simulink model "sc_1"  (R2024b)
settings: Solver=VariableStepAuto  StartTime=0.0  StopTime=10.0  RelTol=1e-3
settings Model: Creator=alex_  LastModifiedBy=alex_

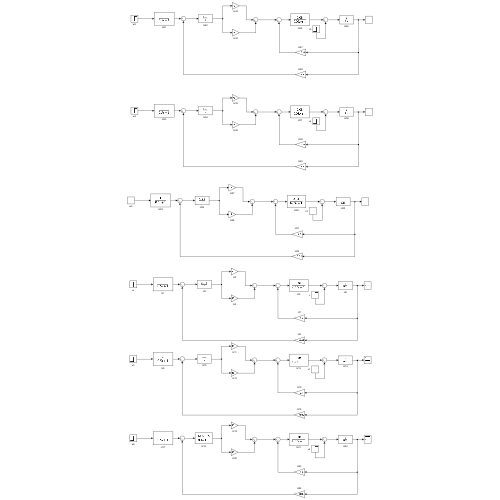
[thumbnail: Simulink's stored preview of the top-level diagram]
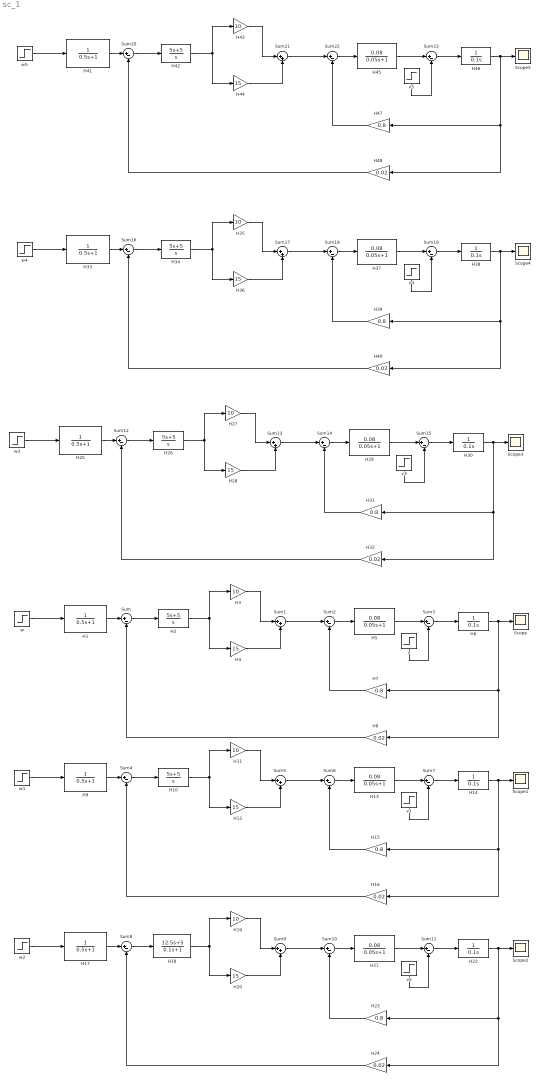
== system sc_1 ==
  H{1,9,17,25,33,41} (6 alike) : TransferFcn  Denominator=[0.5 1]
  H{2,10,26,34,42} (5 alike) : TransferFcn  Numerator=[5 5]  Denominator=[1 0]
  H{3,11,19,27,35,43} (6 alike) : Gain  Gain=10
  H{4,12,20,28,36,44} (6 alike) : Gain  Gain=15
  H{5,13,21,29,37,45} (6 alike) : TransferFcn  Numerator=[0.08]  Denominator=[0.05 1]
  H{6,14,22,30,38,46} (6 alike) : TransferFcn  Denominator=[0.1 0]
  H{7,15,23,31,39,47} (6 alike) : Gain  Gain=0.8
  H{8,16,24,32,40,48} (6 alike) : Gain  Gain=0.02
  H18 : TransferFcn  Numerator=[12.5 5]  Denominator=[0.1 1]
  Scope{,1..5} (6 alike) : Scope
  Sum{,2..4,6..8,10..12,14..16,18..20,22..23} (18 alike) : Sum  Inputs=|+-
  Sum{1,5,9,13,17,21} (6 alike) : Sum  Inputs=|++
  v : Step  Time=0  After=5  SampleTime=0
  v1 : Step  Time=0  After=10  SampleTime=0
  v2 : Step  Time=0  After=5  SampleTime=0
  v3 : Step  Time=0  After=0  SampleTime=0
  v4 : Step  Time=0  After=0  SampleTime=0
  v5 : Step  Time=0  After=0  SampleTime=0
  w{,1..3} (4 alike) : Step  Time=0  After=6  SampleTime=0
  w4 : Step  Time=0  After=3  SampleTime=0
  w5 : Step  Time=0  After=0  SampleTime=0
  wires:
  w/1 -> H1/1
  H1/1 -> Sum/1
  Sum/1 -> H2/1
  H2/1 -> H4/1, H3/1
  H3/1 -> Sum1/1
  H4/1 -> Sum1/2
  Sum1/1 -> Sum2/1
  Sum2/1 -> H5/1
  H5/1 -> Sum3/1
  Sum3/1 -> H6/1
  v/1 -> Sum3/2
  H6/1 -> Scope/1, H8/1, H7/1
  H7/1 -> Sum2/2
  H8/1 -> Sum/2
  H14/1 -> Scope1/1, H16/1, H15/1
  Sum7/1 -> H14/1
  Sum5/1 -> Sum6/1
  Sum6/1 -> H13/1
  H15/1 -> Sum6/2
  H10/1 -> H12/1, H11/1
  H13/1 -> Sum7/1
  H16/1 -> Sum4/2
  v1/1 -> Sum7/2
  H12/1 -> Sum5/2
  H11/1 -> Sum5/1
  w1/1 -> H9/1
  Sum4/1 -> H10/1
  H9/1 -> Sum4/1
  H22/1 -> Scope2/1, H24/1, H23/1
  Sum11/1 -> H22/1
  Sum9/1 -> Sum10/1
  Sum10/1 -> H21/1
  H23/1 -> Sum10/2
  H18/1 -> H20/1, H19/1
  H21/1 -> Sum11/1
  H24/1 -> Sum8/2
  v2/1 -> Sum11/2
  H20/1 -> Sum9/2
  H19/1 -> Sum9/1
  w2/1 -> H17/1
  Sum8/1 -> H18/1
  H17/1 -> Sum8/1
  H30/1 -> Scope3/1, H32/1, H31/1
  Sum15/1 -> H30/1
  Sum13/1 -> Sum14/1
  Sum14/1 -> H29/1
  H31/1 -> Sum14/2
  H26/1 -> H28/1, H27/1
  H29/1 -> Sum15/1
  H32/1 -> Sum12/2
  v3/1 -> Sum15/2
  H28/1 -> Sum13/2
  H27/1 -> Sum13/1
  w3/1 -> H25/1
  Sum12/1 -> H26/1
  H25/1 -> Sum12/1
  H38/1 -> Scope4/1, H40/1, H39/1
  Sum19/1 -> H38/1
  Sum17/1 -> Sum18/1
  Sum18/1 -> H37/1
  H39/1 -> Sum18/2
  H34/1 -> H36/1, H35/1
  H37/1 -> Sum19/1
  H40/1 -> Sum16/2
  v4/1 -> Sum19/2
  H36/1 -> Sum17/2
  H35/1 -> Sum17/1
  w4/1 -> H33/1
  Sum16/1 -> H34/1
  H33/1 -> Sum16/1
  H46/1 -> Scope5/1, H48/1, H47/1
  Sum23/1 -> H46/1
  Sum21/1 -> Sum22/1
  Sum22/1 -> H45/1
  H47/1 -> Sum22/2
  H42/1 -> H44/1, H43/1
  H45/1 -> Sum23/1
  H48/1 -> Sum20/2
  v5/1 -> Sum23/2
  H44/1 -> Sum21/2
  H43/1 -> Sum21/1
  w5/1 -> H41/1
  Sum20/1 -> H42/1
  H41/1 -> Sum20/1
